simulink model "MECC_DCMotor_Pendulum"  (R2026a)
settings: Solver=FixedStepDiscrete  StopTime=inf  FixedStep=.01
undefined symbols (not defined in the file or in its folder): kd, ki, kp
libraries: sl_discontinuities x4, arduinolib x3, simulink x2, arduinosensorlib x1
settings Model: SimulationMode=external  SILPILModeSetting=veronly  ExtModeTrigDuration=2  Creator=thomp  LastModifiedBy=atekes
settings HardwareCC: ProdBitPerInt=16.0  ProdBitPerPointer=16.0  ProdBitPerSizeT=16.0  ProdBitPerPtrDiffT=16.0  ProdWordSize=8.0  ProdHWDeviceType=Atmel->AVR
settings RTWCC: SystemTargetFile=ert.tlc  HardwareBoard=Arduino Uno  TLCOptions=-aInlineSetEventsForThisBaseRateFcn=TLC_FALSE -aSuppressMultiTaskScheduler=TLC_FALSE -aRateBasedStepFcn=1  Toolchain=Arduino AVR  BuildConfiguration=Faster Runs  Description=Embedded Coder
settings ERTTargetCC: ExtModeTransport=3.0  ExtModeAutomaticAllocSize=off  ExtModeStaticAllocSize=250.0  SupportContinuousTime=on  SupportVariableSizeSignals=on

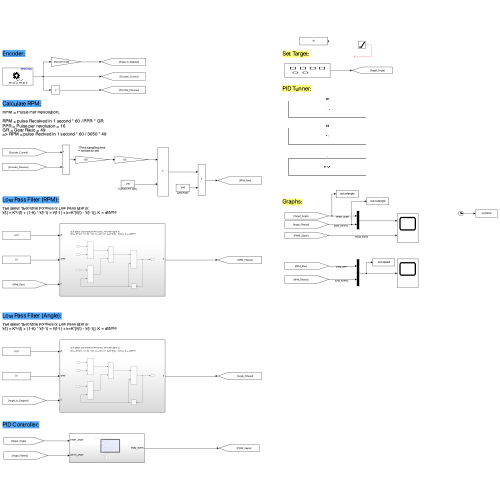
[thumbnail: Simulink's stored preview of the top-level diagram]
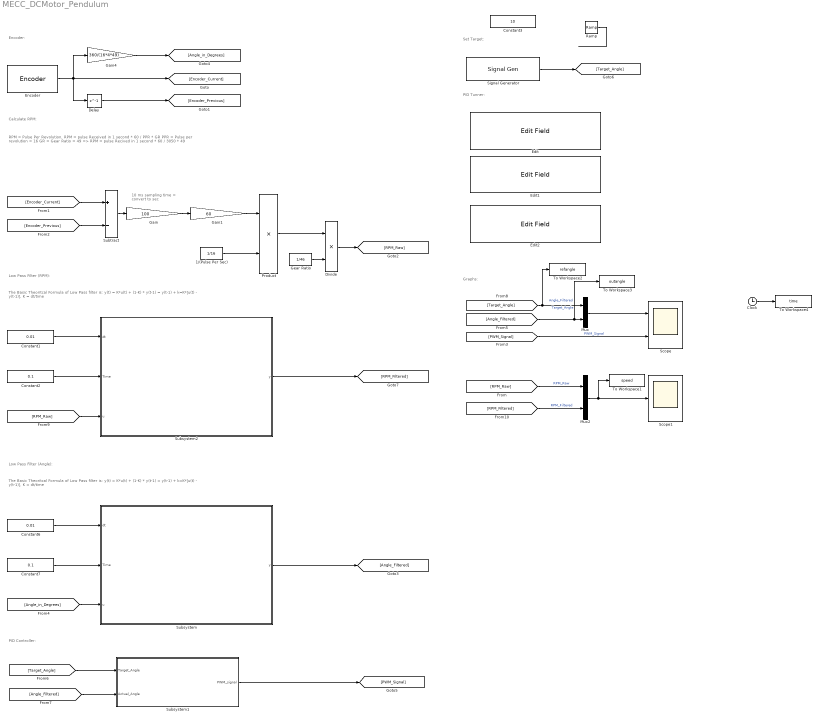
== system MECC_DCMotor_Pendulum ==
  note: 10 ms sampling time = convert to sec
  note: The Basic Theoritcal Formula of Low Pass filter is:
      | y(t) = K*u(t) + (1-K) * y(t-1) = y(t-1) + k=K*[u(t) - y(t-1)], K = dt/time
  note: RPM = Pulse Per Revolution,
      |
      | RPM = pulse Received in 1 second * 60 / PPR * GR
      | PPR = Pulse per revolution = 16
      | GR = Gear Ratio = 49
      | => RPM = pulse Recived in 1 second * 60 / 3050 * 49
  note: PID Tunner:
  note: Encoder:
  note: Calculate RPM:
  note: Low Pass Filter (Angle):
  note: PID Controller:
  note: Set Target:
  note: The Basic Theoritcal Formula of Low Pass filter is:
      | y(t) = K*u(t) + (1-K) * y(t-1) = y(t-1) + k=K*[u(t) - y(t-1)], K = dt/time
  note: Low Pass Filter (RPM):
  note: Graphs:
  1/(Pulse Per Sec) : Constant  Value=1/16
  Clock : Clock
  Constant1 : Constant  Value=0.01
  Constant2 : Constant  Value=0.1
  Constant3 : Constant  Value=10
  Constant6 : Constant  Value=0.01
  Constant7 : Constant  Value=0.1
  Delay : Delay  DelayLength=1
  Divide : Product  Inputs=**
  Edit : EditField  ShowInitialText=on  Alignment=Center
  Edit1 : EditField  ShowInitialText=on  Alignment=Center
  Edit2 : EditField  ShowInitialText=on  Alignment=Center
  Encoder : arduinosensorlib/Encoder  InputA=2  InputB=3  Mode=No reset  SampleTime=-1
  Gain : Gain  Gain=100
  Gain1 : Gain  Gain=60
  Gain4 : Gain  Gain=360/(16*4*49)
  Gear Ratio : Constant  Value=1/46
  Mux : Mux  Inputs=2
  Mux2 : Mux  Inputs=2
  Product : Product
  Ramp : simulink/Sources/Ramp  slope=5000  start=0  InitialOutput=0
  Scope : Scope  NumInputPorts=2
      settings: ActiveDisplayYMinimum=-72  ActiveDisplayYMaximum=72
  Scope1 : Scope
      settings: ActiveDisplayYMinimum=-800  ActiveDisplayYMaximum=800
  Signal Generator : SignalGenerator  WaveForm=square  Amplitude=45  Frequency=2*pi/8  Units=rad/sec
  Subsystem : Subsystem
  Subsystem1 : Subsystem
  Subsystem2 : Subsystem
  Subtract : Sum  Inputs=+-
  To Workspace1 : ToWorkspace  VariableName=speed  SampleTime=-1
  To Workspace2 : ToWorkspace  VariableName=refangle  SampleTime=-1
  To Workspace3 : ToWorkspace  VariableName=outangle  SampleTime=-1
  To Workspace4 : ToWorkspace  VariableName=time  SampleTime=-1
  wires:
  [Encoder_Current] -> Subtract/1
  [Encoder_Previous] -> Subtract/2
  Subtract/1 -> Gain/1
  Gain/1 -> Gain1/1
  Gain1/1 -> Product/1
  1/(Pulse Per Sec)/1 -> Product/2
  Product/1 -> Divide/1
  Divide/1 -> [RPM_Raw]
  [Angle_in_Degrees] -> Subsystem/3(u)
  Constant6/1 -> Subsystem/1(dt)
  Constant7/1 -> Subsystem/2(Time)
  Subsystem/1(y) -> [Angle_Filtered]
  [Angle_Filtered] -> To Workspace3/1, Mux/2  "Angle_Filtered"
  Delay/1 -> [Encoder_Previous]
  Encoder/1 -> [Encoder_Current], Gain4/1, Delay/1
  Gain4/1 -> [Angle_in_Degrees]
  [Angle_Filtered] -> Subsystem1/2(Actual_Angle)
  Subsystem1/1(PWM_signal) -> [PWM_Signal]
  [Target_Angle] -> Subsystem1/1(Target_Angle)
  [Target_Angle] -> To Workspace2/1, Mux/1  "Target_Angle"
  Mux/1 -> Scope/1
  [PWM_Signal] -> Scope/2  "PWM_Signal"
  [RPM_Raw] -> Mux2/1  "RPM_Raw"
  Subsystem2/1(y) -> [RPM_Filtered]
  Constant2/1 -> Subsystem2/2(Time)
  Constant1/1 -> Subsystem2/1(dt)
  [RPM_Raw] -> Subsystem2/3(u)
  [RPM_Filtered] -> Mux2/2  "RPM_Filtered"
  Mux2/1 -> To Workspace1/1, Scope1/1
  Gear Ratio/1 -> Divide/2
  Ramp/1 -> ?
  Signal Generator/1 -> [Target_Angle]
  Clock/1 -> To Workspace4/1

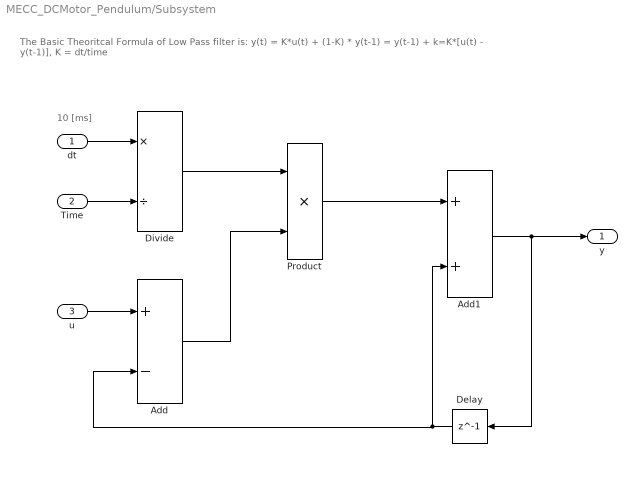
== system MECC_DCMotor_Pendulum/Subsystem ==
  note: 10 [ms]
  note: The Basic Theoritcal Formula of Low Pass filter is:
      | y(t) = K*u(t) + (1-K) * y(t-1) = y(t-1) + k=K*[u(t) - y(t-1)], K = dt/time
  dt : Inport
  Time : Inport  Port=2
  u : Inport  Port=3
  Add : Sum  Inputs=+-
  Add1 : Sum
  Delay : Delay  DelayLength=1
  Divide : Product  Inputs=*/
  Product : Product
  y : Outport
  wires:
  dt/1 -> Divide/1
  Time/1 -> Divide/2
  u/1 -> Add/1
  Add/1 -> Product/2
  Divide/1 -> Product/1
  Product/1 -> Add1/1
  Add1/1 -> Delay/1, y/1
  Delay/1 -> Add1/2, Add/2

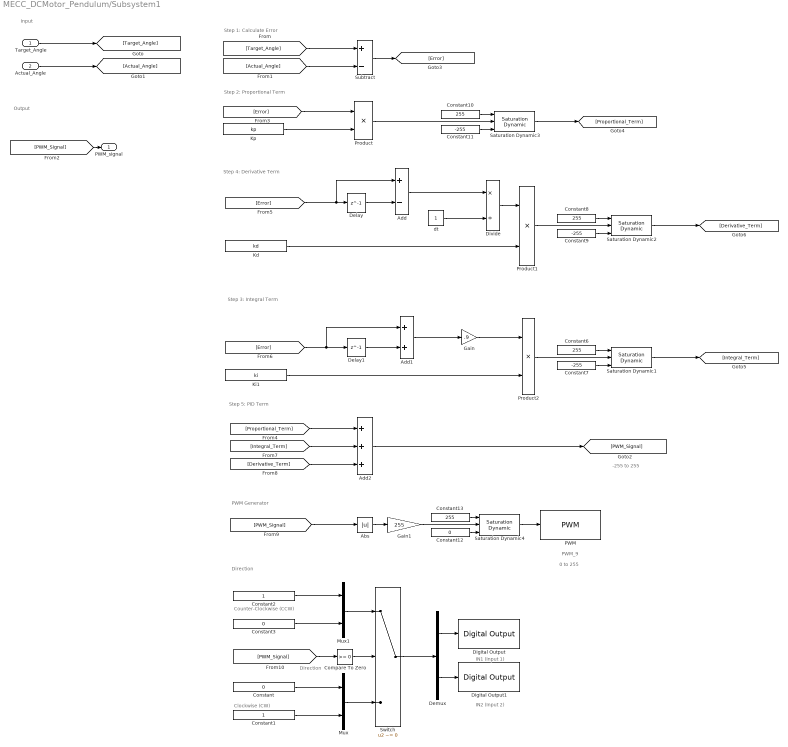
== system MECC_DCMotor_Pendulum/Subsystem1 ==
  note: -255 to 255
  note: Step 1: Calculate Error
  note: Input
  note: Output
  note: Step 2: Proportional Term
  note: Step 3: Integral Term
  note: Step 4: Derivative Term
  note: Step 5: PID Term
  note: PWM Generator
  note: PWM_9
  note: 0 to 255
  note: Direction
  note: Direction
  note: Counter-Clockwise (CCW)
  note: Clockwise (CW)
  note: IN2 (Input 2)
  note: IN1 (Input 1)
  Target_Angle : Inport
  Actual_Angle : Inport  Port=2
  Abs : Abs  SaturateOnIntegerOverflow=off
  Add : Sum  Inputs=+-
  Add1 : Sum
  Add2 : Sum  Inputs=+++
  Compare To Zero : simulink/Logic and Bit Operations/Compare To Zero  relop=>=  OutDataTypeStr=boolean
  Constant : Constant  Value=0  OutMin=0  OutMax=1  OutDataTypeStr=uint8
  Constant1 : Constant  OutMin=0  OutMax=1  OutDataTypeStr=uint8
  Constant{6,8,10,13} (4 alike) : Constant  Value=255
  Constant11 : Constant  Value=-255
  Constant12 : Constant  Value=0
  Constant2 : Constant  OutMin=0  OutMax=1  OutDataTypeStr=uint8
  Constant3 : Constant  Value=0  OutMin=0  OutMax=1  OutDataTypeStr=uint8
  Constant7 : Constant  Value=-255
  Constant9 : Constant  Value=-255
  Delay : Delay  DelayLength=1  InputProcessing=Columns as channels (frame based)
  Delay1 : Delay  DelayLength=1  InputProcessing=Columns as channels (frame based)
  Demux : Demux  Outputs=2
  Digital Output : arduinolib/Digital Output  pinNumber=7  Direction=output  blockPlatform=arduino
  Digital Output1 : arduinolib/Digital Output  pinNumber=8  Direction=output  blockPlatform=arduino
  Divide : Product  Inputs=*/
  Gain : Gain  Gain=.9
  Gain1 : Gain  Gain=255
  Kd : Constant  Value=kd
  Ki1 : Constant  Value=ki
  Kp : Constant  Value=kp
  Mux : Mux  Inputs=2
  Mux1 : Mux  Inputs=2
  PWM : arduinolib/PWM  pinNumber=9  frequencyType=Default  desiredFrequency=490.2  achievableFrequency=490.2
  Product : Product
  Product1 : Product
  Product2 : Product
  Saturation Dynamic{1..4} (4 alike) : sl_discontinuities/Saturation Dynamic  OutMin=[]  OutMax=[]  OutDataTypeStr=Inherit: Same as second input  OutDataType=fixdt(1, 16)  OutScaling=2^-10  DoSatur=off
  Subtract : Sum  Inputs=+-
  Switch : Switch  Criteria=u2 ~= 0  SaturateOnIntegerOverflow=off  InputSameDT=off
  dt : Constant
  PWM_signal : Outport
  wires:
  Target_Angle/1 -> [Target_Angle]
  Actual_Angle/1 -> [Actual_Angle]
  [PWM_Signal] -> PWM_signal/1
  [Target_Angle] -> Subtract/1
  [Actual_Angle] -> Subtract/2
  Subtract/1 -> [Error]
  [Error] -> Product/1
  Kp/1 -> Product/2
  [Error] -> Delay/1, Add/1
  Product2/1 -> Saturation Dynamic1/2
  [Error] -> Add1/1, Delay1/1
  Ki1/1 -> Product2/2
  [Proportional_Term] -> Add2/1
  [Derivative_Term] -> Add2/3
  [Integral_Term] -> Add2/2
  Gain1/1 -> Saturation Dynamic4/2
  [PWM_Signal] -> Abs/1
  Abs/1 -> Gain1/1
  [PWM_Signal] -> Compare To Zero/1
  Mux/1 -> Switch/3
  Mux1/1 -> Switch/1
  Switch/1 -> Demux/1
  Constant1/1 -> Mux/2
  Constant/1 -> Mux/1
  Demux/2 -> Digital Output1/1
  Demux/1 -> Digital Output/1
  Compare To Zero/1 -> Switch/2
  Constant2/1 -> Mux1/1
  Constant3/1 -> Mux1/2
  Add2/1 -> [PWM_Signal]
  Constant7/1 -> Saturation Dynamic1/3
  Constant6/1 -> Saturation Dynamic1/1
  Saturation Dynamic1/1 -> [Integral_Term]
  Constant8/1 -> Saturation Dynamic2/1
  Constant9/1 -> Saturation Dynamic2/3
  Product1/1 -> Saturation Dynamic2/2
  Saturation Dynamic2/1 -> [Derivative_Term]
  Product/1 -> Saturation Dynamic3/2
  Constant11/1 -> Saturation Dynamic3/3
  Constant10/1 -> Saturation Dynamic3/1
  Saturation Dynamic3/1 -> [Proportional_Term]
  Delay/1 -> Add/2
  Add/1 -> Divide/1
  dt/1 -> Divide/2
  Divide/1 -> Product1/1
  Kd/1 -> Product1/2
  Delay1/1 -> Add1/2
  Add1/1 -> Gain/1
  Gain/1 -> Product2/1
  Saturation Dynamic4/1 -> PWM/1
  Constant12/1 -> Saturation Dynamic4/3
  Constant13/1 -> Saturation Dynamic4/1

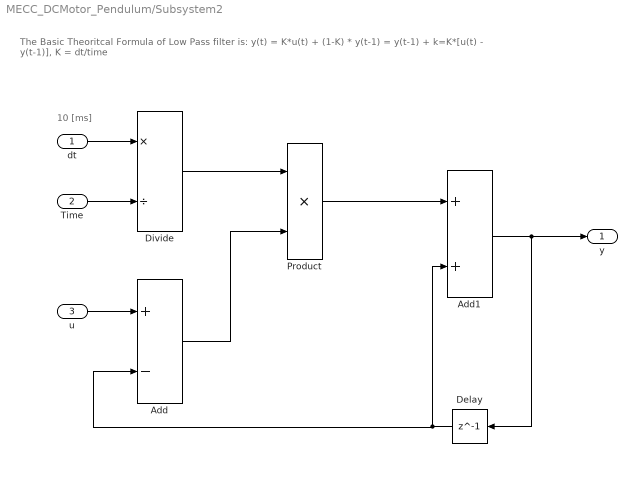
== system MECC_DCMotor_Pendulum/Subsystem2 ==
  note: The Basic Theoritcal Formula of Low Pass filter is:
      | y(t) = K*u(t) + (1-K) * y(t-1) = y(t-1) + k=K*[u(t) - y(t-1)], K = dt/time
  note: 10 [ms]
  dt : Inport
  Time : Inport  Port=2
  u : Inport  Port=3
  Add : Sum  Inputs=+-
  Add1 : Sum
  Delay : Delay  DelayLength=1
  Divide : Product  Inputs=*/
  Product : Product
  y : Outport
  wires:
  Delay/1 -> Add/2, Add1/2
  Add1/1 -> y/1, Delay/1
  Product/1 -> Add1/1
  Divide/1 -> Product/1
  Add/1 -> Product/2
  u/1 -> Add/1
  Time/1 -> Divide/2
  dt/1 -> Divide/1
